simulink model "FMS1"  (R2018b)
settings: configuration reference "fms_config" (kept outside this file)
values from neighbouring files (symbols this model uses):
  FMS_EXPORT = Simulink.Parameter(FMS_EXPORT_VALUE)    [fms_model_init.m]
  FMS_PARAM = Simulink.Parameter(FMS_PARAM_VALUE)    [fms_model_init.m]
undefined symbols (not defined in the file or in its folder): actuator_cmd, ax_cmd, ay_cmd, az_cmd, cmd_mask, ControlMode, ctrl_mode, DiscIntNeverNeededParam, FMS_Cmd, FMS_CONST, home, mode, p_cmd, phi_cmd, PilotMode, psi_rate_cmd, q_cmd, r_cmd, reset, state, status, theta_cmd, throttle_cmd, timestamp, u_cmd, v_cmd, VehicleState, VehicleStatus, w_cmd, wp_consume, wp_current
libraries: simulink x119, FMT_Model_Lib x56, hdlsllib x13
(part 4 of 7)

== system FMS1/FMS Commander/Commander/Arm/Assist/Position/Position Command/Controller/Hold Control ==
  FMS_In : Inport
  Action Port : ActionPort  InitializeStates=reset  ActionType=case
  Bus Selector : BusSelector  OutputSignals=INS_Out.psi
  Bus_Selection : Subsystem
  Constant : Constant  Value=0  OutDataTypeStr=Inherit: Inherit via back propagation
  Delay : Delay  DelayLength=1  InitialConditionSource=Input port
      settings: InputPortMap=u0,p4
  Gain2 : Gain  Gain=FMS_PARAM.XY_P  OutDataTypeStr=single
  Multiply : Product  Multiplication=Matrix(*)
  Mux : Mux  Inputs=2
  Psi To DCM : FMT_Model_Lib/Transformation/Psi To DCM
      settings: SourceProductName=FMT Toolbox
  Selector : Selector  InputPortWidth=3  IndexOptions=Index vector (dialog)  Indices=[1 2]  OutputSizes=1
  Sum : Sum  Inputs=-+|
  uv_cmd_mPs : Outport
  wires:
  Bus Selector/1 -> Psi To DCM/1  "<psi>"
  Selector/1 -> Gain2/1
  Mux/1 -> Multiply/2
  Multiply/1 -> Selector/1
  Psi To DCM/1 -> Multiply/1  "M_CO"
  Constant/1 -> Mux/2
  FMS_In/1 -> Bus_Selection/1(FMS_In), Bus Selector/1
  Delay/1 -> Sum/2, Delay/1  "xy_cmd_R"
  Sum/1 -> Mux/1  "xy_err_R"
  Bus_Selection/1(xy_R_O_m) -> Delay/2, Sum/1  "xy_est_R"
  Gain2/1 -> uv_cmd_mPs/1

== system FMS1/FMS Commander/Commander/Arm/Assist/Position/Position Command/Controller/Move Control ==
  FMS_In : Inport
  Action Port : ActionPort  InitializeStates=reset  ActionType=case
  Bus Selector : BusSelector  OutputSignals=Pilot_Cmd.stick_pitch,Pilot_Cmd.stick_roll
  Compare To Constant : simulink/Logic and Bit Operations/Compare To Constant  relop=>  const=1  OutDataTypeStr=boolean
  DeadZone : Subsystem  mask{th=FMS_PARAM.PITCH_DZ}
      mask prompts: th "Threshold"
      mask Display: disp('Dead Zone')
  DeadZone1 : Subsystem  mask{th=FMS_PARAM.ROLL_DZ}
      mask prompts: th "Threshold"
      mask Display: disp('Dead Zone')
  Gain6 : Gain  Gain=FMS_PARAM.VEL_XY_LIM  OutDataTypeStr=single
  Mux1 : Mux  Inputs=2
  Switch : Switch  Criteria=u2 > Threshold
  TD : Subsystem
  Vector Modulus : FMT_Model_Lib/Math/Vector Modulus
      settings: SourceProductName=FMT Toolbox
  Vector Normalize : FMT_Model_Lib/Math/Vector Normalize
      settings: SourceProductName=FMT Toolbox
  uv_cmd_mPs : Outport
  wires:
  DeadZone1/1(y) -> Mux1/2
  Bus Selector/2 -> DeadZone1/1(u)  "<stick_roll>"
  TD/1(v1) -> uv_cmd_mPs/1
  FMS_In/1 -> Bus Selector/1
  Bus Selector/1 -> DeadZone/1(u)  "<stick_pitch>"
  DeadZone/1(y) -> Mux1/1
  Gain6/1 -> TD/1(v)
  Switch/1 -> Gain6/1
  Mux1/1 -> Switch/3, Vector Normalize/1, Vector Modulus/1
  Vector Modulus/1 -> Compare To Constant/1
  Compare To Constant/1 -> Switch/2
  Vector Normalize/1 -> Switch/1

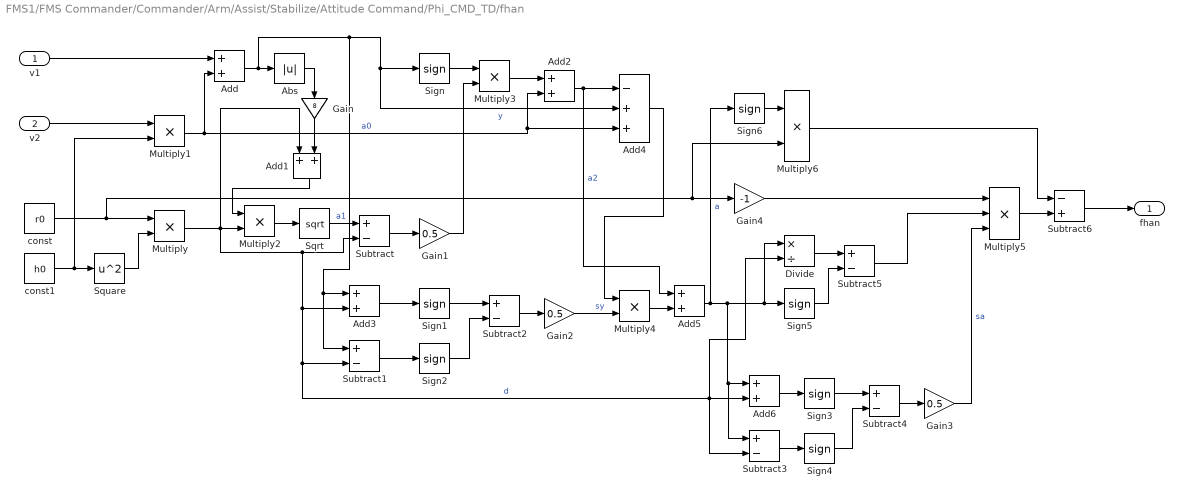
== system FMS1/FMS Commander/Commander/Arm/Assist/Stabilize/Attitude Command/Phi_CMD_TD/fhan  ==
  v1 : Inport
  v2 : Inport  Port=2
  Abs : Abs
  Add{,1..3,5..6} (6 alike) : Sum  OutDataTypeStr=Inherit: Same as first input
  Add4 : Sum  Inputs=-++
  Divide : Product  Inputs=*/
  Gain : Gain  Gain=8
  Gain1 : Gain  Gain=0.5  OutDataTypeStr=Inherit: Same as input
  Gain2 : Gain  Gain=0.5  OutDataTypeStr=Inherit: Same as input
  Gain3 : Gain  Gain=0.5  OutDataTypeStr=Inherit: Same as input
  Gain4 : Gain  Gain=-1  OutDataTypeStr=Inherit: Same as input
  Multiply{,1..3} (4 alike) : Product  OutDataTypeStr=Inherit: Same as first input
  Multiply4 : Product  OutDataTypeStr=single
  Multiply5 : Product  Inputs=3
  Multiply6 : Product  OutDataTypeStr=single
  Sign{,1..6} (7 alike) : Signum
  Sqrt : Sqrt  SaturateOnIntegerOverflow=on
  Square : Math  Operator=square  SaturateOnIntegerOverflow=on
  Subtract{,1..5} (6 alike) : Sum  Inputs=+-  OutDataTypeStr=Inherit: Same as first input
  Subtract6 : Sum  Inputs=-+  OutDataTypeStr=Inherit: Same as first input
  const : Constant  Value=r0  OutDataTypeStr=single
  const1 : Constant  Value=h0  OutDataTypeStr=single
  fhan : Outport
  wires:
  v1/1 -> Add/1
  Sign/1 -> Multiply3/1
  Gain2/1 -> Multiply4/2  "sy"
  v2/1 -> Multiply1/1
  Gain3/1 -> Multiply5/3  "sa"
  Subtract/1 -> Gain1/1
  Subtract6/1 -> fhan/1
  Sign2/1 -> Subtract2/2
  Sign4/1 -> Subtract4/2
  Abs/1 -> Gain/1
  Add4/1 -> Multiply4/1
  Sign5/1 -> Subtract5/2
  Sqrt/1 -> Subtract/1  "a1"
  Subtract3/1 -> Sign4/1
  Add1/1 -> Multiply2/1
  Subtract1/1 -> Sign2/1
  Divide/1 -> Subtract5/1
  Multiply3/1 -> Add2/1
  Gain/1 -> Add1/2
  const/1 -> Multiply6/2, Gain4/1, Multiply/1
  Add3/1 -> Sign1/1
  Subtract5/1 -> Multiply5/2
  Multiply4/1 -> Add5/2
  const1/1 -> Multiply1/2, Square/1
  Add5/1 -> Sign6/1, Sign5/1, Divide/1, Subtract3/1, Add6/1  "a"
  Multiply1/1 -> Add4/3, Add2/2, Add/2  "a0"
  Add/1 -> Subtract1/1, Add3/1, Add4/2, Sign/1, Abs/1  "y"
  Subtract2/1 -> Gain2/1
  Add2/1 -> Add4/1, Add5/1  "a2"
  Subtract4/1 -> Gain3/1
  Gain4/1 -> Multiply5/1
  Multiply5/1 -> Subtract6/2
  Sign6/1 -> Multiply6/1
  Sign3/1 -> Subtract4/1
  Add6/1 -> Sign3/1
  Multiply/1 -> Subtract/2, Divide/2, Subtract3/2, Add6/2, Subtract1/2, Add3/2, Add1/1, Multiply2/2  "d"
  Multiply6/1 -> Subtract6/1
  Gain1/1 -> Multiply3/2
  Square/1 -> Multiply/2
  Multiply2/1 -> Sqrt/1
  Sign1/1 -> Subtract2/1

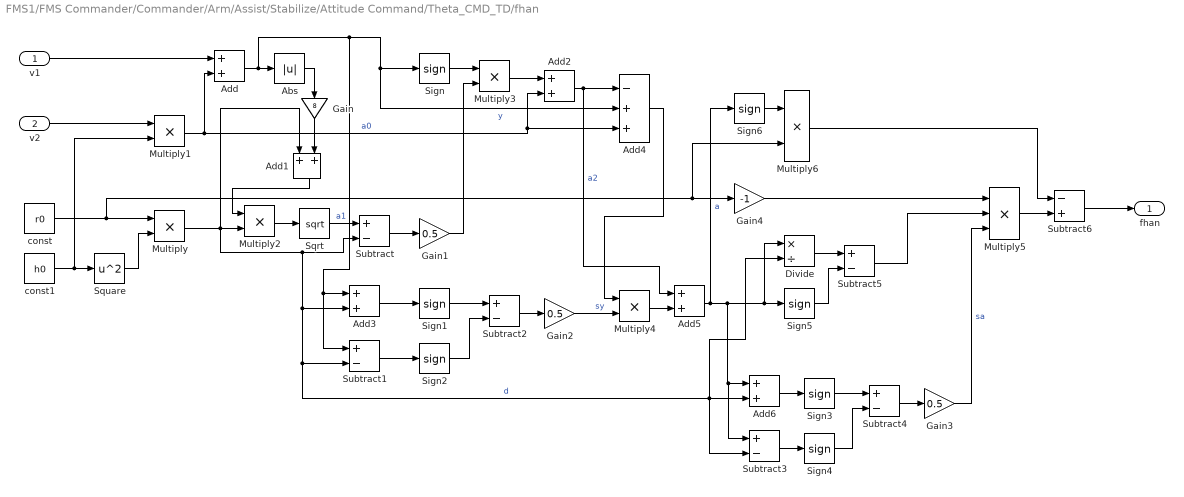
== system FMS1/FMS Commander/Commander/Arm/Assist/Stabilize/Attitude Command/Theta_CMD_TD/fhan  ==
  v1 : Inport
  v2 : Inport  Port=2
  Abs : Abs
  Add{,1..3,5..6} (6 alike) : Sum  OutDataTypeStr=Inherit: Same as first input
  Add4 : Sum  Inputs=-++
  Divide : Product  Inputs=*/
  Gain : Gain  Gain=8
  Gain1 : Gain  Gain=0.5  OutDataTypeStr=Inherit: Same as input
  Gain2 : Gain  Gain=0.5  OutDataTypeStr=Inherit: Same as input
  Gain3 : Gain  Gain=0.5  OutDataTypeStr=Inherit: Same as input
  Gain4 : Gain  Gain=-1  OutDataTypeStr=Inherit: Same as input
  Multiply{,1..3} (4 alike) : Product  OutDataTypeStr=Inherit: Same as first input
  Multiply4 : Product  OutDataTypeStr=single
  Multiply5 : Product  Inputs=3
  Multiply6 : Product  OutDataTypeStr=single
  Sign{,1..6} (7 alike) : Signum
  Sqrt : Sqrt  SaturateOnIntegerOverflow=on
  Square : Math  Operator=square  SaturateOnIntegerOverflow=on
  Subtract{,1..5} (6 alike) : Sum  Inputs=+-  OutDataTypeStr=Inherit: Same as first input
  Subtract6 : Sum  Inputs=-+  OutDataTypeStr=Inherit: Same as first input
  const : Constant  Value=r0  OutDataTypeStr=single
  const1 : Constant  Value=h0  OutDataTypeStr=single
  fhan : Outport
  wires:
  v1/1 -> Add/1
  Sign/1 -> Multiply3/1
  Gain2/1 -> Multiply4/2  "sy"
  v2/1 -> Multiply1/1
  Gain3/1 -> Multiply5/3  "sa"
  Subtract/1 -> Gain1/1
  Subtract6/1 -> fhan/1
  Sign2/1 -> Subtract2/2
  Sign4/1 -> Subtract4/2
  Abs/1 -> Gain/1
  Add4/1 -> Multiply4/1
  Sign5/1 -> Subtract5/2
  Sqrt/1 -> Subtract/1  "a1"
  Subtract3/1 -> Sign4/1
  Add1/1 -> Multiply2/1
  Subtract1/1 -> Sign2/1
  Divide/1 -> Subtract5/1
  Multiply3/1 -> Add2/1
  Gain/1 -> Add1/2
  const/1 -> Multiply6/2, Gain4/1, Multiply/1
  Add3/1 -> Sign1/1
  Subtract5/1 -> Multiply5/2
  Multiply4/1 -> Add5/2
  const1/1 -> Multiply1/2, Square/1
  Add5/1 -> Sign6/1, Sign5/1, Divide/1, Subtract3/1, Add6/1  "a"
  Multiply1/1 -> Add4/3, Add2/2, Add/2  "a0"
  Add/1 -> Subtract1/1, Add3/1, Add4/2, Sign/1, Abs/1  "y"
  Subtract2/1 -> Gain2/1
  Add2/1 -> Add4/1, Add5/1  "a2"
  Subtract4/1 -> Gain3/1
  Gain4/1 -> Multiply5/1
  Multiply5/1 -> Subtract6/2
  Sign6/1 -> Multiply6/1
  Sign3/1 -> Subtract4/1
  Add6/1 -> Sign3/1
  Multiply/1 -> Subtract/2, Divide/2, Subtract3/2, Add6/2, Subtract1/2, Add3/2, Add1/1, Multiply2/2  "d"
  Multiply6/1 -> Subtract6/1
  Gain1/1 -> Multiply3/2
  Square/1 -> Multiply/2
  Multiply2/1 -> Sqrt/1
  Sign1/1 -> Subtract2/1

== system FMS1/FMS Commander/Commander/Arm/Assist/Stabilize/Heading Command/Controller/Brake Control ==
  Action Port : ActionPort  InitializeStates=reset  ActionType=case
  Brake Speed : Constant  Value=0  VectorParams1D=off  OutDataTypeStr=single
  psi_rate_cmd_radPs : Outport
  wires:
  Brake Speed/1 -> psi_rate_cmd_radPs/1

== system FMS1/FMS Commander/Commander/Arm/Assist/Stabilize/Heading Command/Controller/Hold Control ==
  FMS_In : Inport
  Action Port : ActionPort  InitializeStates=reset  ActionType=case
  Bus_Selection : Subsystem
  Delay : Delay  DelayLength=1  InitialConditionSource=Input port
      settings: InputPortMap=u0,p4
  Gain2 : Gain  Gain=FMS_PARAM.YAW_P  OutDataTypeStr=single
  Sum : Sum  Inputs=-+|
  psi_err_saturation : Subsystem
  psi_rate_cmd_radPs : Outport
  wires:
  Gain2/1 -> psi_rate_cmd_radPs/1
  FMS_In/1 -> Bus_Selection/1(FMS_In)
  Delay/1 -> Sum/2, Delay/1  "psi_cmd_rad"
  Sum/1 -> psi_err_saturation/1(psi_err_in)  "psi_error_rad"
  psi_err_saturation/1(psi_err_rad) -> Gain2/1
  Bus_Selection/1(psi_rad) -> Delay/2, Sum/1  "psi_est_rad"

== system FMS1/FMS Commander/Commander/Arm/Assist/Stabilize/Heading Command/Controller/Move Control ==
  FMS_In : Inport
  Action Port : ActionPort  InitializeStates=reset  ActionType=case
  Bus Selector : BusSelector  OutputSignals=Pilot_Cmd.stick_yaw
  DeadZone : Subsystem  mask{th=FMS_PARAM.YAW_DZ}
      mask prompts: th "Threshold"
      mask Display: disp('Dead Zone')
  Gain1 : Gain  Gain=FMS_PARAM.YAW_RATE_LIM  OutDataTypeStr=single
  TD : Subsystem
  psi_rate_cmd_radPs : Outport
  wires:
  TD/1(v1) -> psi_rate_cmd_radPs/1
  FMS_In/1 -> Bus Selector/1
  Bus Selector/1 -> DeadZone/1(u)  "<stick_yaw>"
  DeadZone/1(y) -> Gain1/1
  Gain1/1 -> TD/1(v)

== system FMS1/FMS Commander/Commander/Arm/Auto/Mission/Mission_SubSystem/Heading Commander/Heading Control ==
  FMS_In : Inport
  psi_cmd_rad : Inport  Port=2
  Bus Selector : BusSelector  OutputSignals=INS_Out.psi
  Delay : Delay  DelayLength=1  InitialConditionSource=Input port
      settings: InputPortMap=u0,p4
  Heading Control : Subsystem
  Sum : Sum  Inputs=|++
  Sum1 : Sum  Inputs=+-|
  Sum2 : Sum  Inputs=|+-
  TD : Subsystem
  psi_saturation : Subsystem
  psi_saturation1 : Subsystem
  psi_rate_cmd_radPs : Outport
  psi_err_rad : Outport  Port=2
  wires:
  psi_cmd_rad/1 -> Sum2/1, Sum1/1
  Heading Control/1(psi_rate_cmd_radPs) -> psi_rate_cmd_radPs/1
  FMS_In/1 -> Heading Control/1(FMS_In), Bus Selector/1
  TD/1(v1) -> Heading Control/2(psi_cmd_rad)
  Sum1/1 -> psi_saturation1/1(psi_in)
  Bus Selector/1 -> Sum1/2, Delay/2  "<psi>"
  psi_saturation1/1(psi_rad) -> psi_err_rad/1
  Delay/1 -> Delay/1, TD/2(v0), Sum/2, Sum2/2
  Sum2/1 -> psi_saturation/1(psi_in)
  psi_saturation/1(psi_rad) -> Sum/1
  Sum/1 -> TD/1(v)

== system FMS1/FMS Commander/Commander/Arm/Auto/Mission/Mission_SubSystem/Heading Commander/Included Angle ==
  vec1 : Inport
  vec2 : Inport  Port=2
  2D Cross Product : FMT_Model_Lib/Math/2D Cross Product
      settings: SourceProductName=FMT Toolbox
  Acos : Trigonometry  Operator=acos
  Constant4 : Constant  OutDataTypeStr=single
  Demux : Demux  Outputs=2
  Demux1 : Demux  Outputs=2
  Dot Product : DotProduct  InputSameDT=on  OutDataTypeStr=Inherit: Inherit via internal rule
  Multiply : Product
  Mux : Mux  Inputs=2
  Mux1 : Mux  Inputs=2
  Sign1 : Signum
  Switch2 : Switch  Criteria=u2 ~= 0
  Vector Normalize : FMT_Model_Lib/Math/Vector Normalize
      settings: SourceProductName=FMT Toolbox
  Vector Normalize1 : FMT_Model_Lib/Math/Vector Normalize
      settings: SourceProductName=FMT Toolbox
  angle_rad : Outport
  wires:
  Switch2/1 -> Multiply/2
  Acos/1 -> Multiply/1
  Mux/1 -> Vector Normalize1/1
  vec2/1 -> Demux/1
  Constant4/1 -> Switch2/3
  Demux/1 -> Mux/2
  vec1/1 -> Demux1/1
  Multiply/1 -> angle_rad/1
  2D Cross Product/1 -> Sign1/1
  Vector Normalize/1 -> 2D Cross Product/2, Dot Product/1
  Demux/2 -> Mux/1
  Vector Normalize1/1 -> 2D Cross Product/1, Dot Product/2
  Sign1/1 -> Switch2/2, Switch2/1
  Demux1/2 -> Mux1/1
  Mux1/1 -> Vector Normalize/1
  Demux1/1 -> Mux1/2
  Dot Product/1 -> Acos/1

== system FMS1/FMS Commander/Commander/Arm/Auto/Mission/Mission_SubSystem/Velocity Commander/Altitude Control ==
  FMS_In : Inport
  Vg_C_cmd : Inport  Port=2
  Bus Selector3 : BusSelector  OutputSignals=INS_Out.h_R
  Gain : Gain  Gain=FMS_PARAM.Z_P
  Mux : Mux  Inputs=2
  Saturation1 : Saturate  UpperLimit=FMS_PARAM.VEL_Z_LIM  LowerLimit=-FMS_PARAM.VEL_Z_LIM
  Selector : Selector  InputPortWidth=3  IndexOptions=Index vector (dialog)  Indices=[1 2]  OutputSizes=1
  Sum2 : Sum  Inputs=|+-
  Target Height : Subsystem
  vel_C_cmd : Outport
  wires:
  FMS_In/1 -> Bus Selector3/1, Target Height/1(FMS_In)
  Bus Selector3/1 -> Sum2/1  "<h_R>"
  Sum2/1 -> Gain/1
  Gain/1 -> Saturation1/1
  Target Height/1(h_R_sp) -> Sum2/2  "h_R_sp"
  Vg_C_cmd/1 -> Selector/1
  Selector/1 -> Mux/1
  Saturation1/1 -> Mux/2
  Mux/1 -> vel_C_cmd/1

== system FMS1/FMS Commander/Commander/Arm/Auto/Mission/Mission_SubSystem/Velocity Commander/Cruise Speed  ==
  P3 : Inport
  P2 : Inport  Port=2
  set_speed : Inport  Port=3
  rotating : Inport  Port=4
  Acceleration_Speed : DiscreteIntegrator  ExternalReset=level  SampleTime=-1  UpperSaturationLimit=FMS_PARAM.CRUISE_SPEED  LowerSaturationLimit=0  ICPrevOutput=DiscIntNeverNeededParam  ICPrevScaledInput=DiscIntNeverNeededParam
  Compare To Zero : simulink/Logic and Bit Operations/Compare To Zero  relop=>  OutDataTypeStr=boolean
  Constant : Constant  Value=FMS_PARAM.CRUISE_ACC  OutDataTypeStr=single
  Constant1 : Constant  Value=0.5  OutDataTypeStr=single
  Constant2 : Constant  Value=0  OutDataTypeStr=single
  Gain : Gain  Gain=0.5  OutDataTypeStr=Inherit: Same as input
  Saturation Dynamic : simulink/Discontinuities/Saturation Dynamic  OutMin=[]  OutMax=[]  OutDataTypeStr=Inherit: Same as second input  OutDataType=fixdt(1, 16)  OutScaling=2^-10  DoSatur=off
  Saturation Dynamic1 : simulink/Discontinuities/Saturation Dynamic  OutMin=[]  OutMax=[]  OutDataTypeStr=Inherit: Same as second input  OutDataType=fixdt(1, 16)  OutScaling=2^-10  DoSatur=off
  Sum : Sum  Inputs=|+-
  Sum1 : Sum  Inputs=-+|
  Switch : Switch  Criteria=u2 > Threshold  Threshold=FMS_PARAM.L1
  Switch1 : Switch
  Switch2 : Switch  Criteria=u2 > Threshold
  Vector Modulus : FMT_Model_Lib/Math/Vector Modulus
      settings: SourceProductName=FMT Toolbox
  vel : Constant  Value=FMS_PARAM.CRUISE_SPEED  OutDataTypeStr=single
  |Vg| : Outport
  cruise_speed : Outport  Port=2
  wires:
  Gain/1 -> Saturation Dynamic/2
  Switch/1 -> Sum1/1, Switch1/1
  vel/1 -> Switch2/3  "|Vg|"
  Vector Modulus/1 -> Switch/2, Gain/1
  Sum/1 -> Vector Modulus/1
  P2/1 -> Sum/2
  P3/1 -> Sum/1
  Saturation Dynamic/1 -> Switch/3
  Constant/1 -> Acceleration_Speed/1
  Saturation Dynamic1/1 -> Switch1/3, Sum1/2
  Sum1/1 -> Switch1/2
  Switch1/1 -> |Vg|/1
  rotating/1 -> Acceleration_Speed/2
  Switch2/1 -> cruise_speed/1, Saturation Dynamic1/1, Saturation Dynamic/1, Switch/1
  set_speed/1 -> Compare To Zero/1, Switch2/1
  Compare To Zero/1 -> Switch2/2
  Constant1/1 -> Saturation Dynamic/3
  Acceleration_Speed/1 -> Saturation Dynamic1/2
  Constant2/1 -> Saturation Dynamic1/3

== system FMS1/FMS Commander/Commander/Arm/Auto/Mission/Mission_SubSystem/Velocity Commander/Hold Position ==
  FMS_In : Inport
  Altitude Hold : Subsystem
  Mux : Mux  Inputs=3
  Position Hold : Subsystem
  vel_cmd : Outport
  wires:
  FMS_In/1 -> Altitude Hold/1(FMS_In), Position Hold/1(FMS_In)
  Position Hold/2(v_cmd_mPs) -> Mux/2
  Altitude Hold/1(w_cmd_mPs) -> Mux/3
  Position Hold/1(u_cmd_mPs) -> Mux/1
  Mux/1 -> vel_cmd/1

== system FMS1/FMS Commander/Commander/Arm/Auto/Mission/Mission_SubSystem/Velocity Commander/L1 Reference WP ==
  P1 : Inport
  P2 : Inport  Port=2
  P3 : Inport  Port=3
  L1 : Inport  Port=4
  Compare To Constant : simulink/Logic and Bit Operations/Compare To Constant  relop=>=  const=0  OutDataTypeStr=boolean
  Compare To Constant1 : simulink/Logic and Bit Operations/Compare To Constant  relop=>  const=0  OutDataTypeStr=boolean
  NearbyRefWP : MATLAB Function  TreatAsAtomicUnit=on
  OutRegionRegWP : MATLAB Function  TreatAsAtomicUnit=on
  Reshape : Reshape  OutputDimensionality=Customize  OutputDimensions=[2,1]
  SearchL1RefWP : MATLAB Function  TreatAsAtomicUnit=on
  Switch : Switch  Criteria=u2 > Threshold
  Switch1 : Switch  Criteria=u2 > Threshold
  L1_WP : Outport
  wires:
  Reshape/1 -> L1_WP/1
  Compare To Constant/1 -> Switch/2
  NearbyRefWP/2(d) -> Compare To Constant1/1  "distance"
  SearchL1RefWP/2(u) -> Compare To Constant/1  "l1_u"
  Compare To Constant1/1 -> Switch1/2
  P1/1 -> SearchL1RefWP/1(P1), OutRegionRegWP/1(P1)
  P2/1 -> SearchL1RefWP/2(P2), NearbyRefWP/1(P2), OutRegionRegWP/2(P2)
  P3/1 -> NearbyRefWP/2(P3), SearchL1RefWP/3(P3), OutRegionRegWP/3(P3)
  Switch/1 -> Switch1/3
  L1/1 -> SearchL1RefWP/4(L1), NearbyRefWP/3(L1)
  OutRegionRegWP/1(P) -> Switch/3  "out_WP"
  Switch1/1 -> Reshape/1
  SearchL1RefWP/1(P) -> Switch/1  "L1_Ref_P"
  NearbyRefWP/1(P) -> Switch1/1  "NearbyWP"

== system FMS1/FMS Commander/Commander/Arm/Auto/Mission/Mission_SubSystem/Velocity Commander/Lateral Acceleration ==
  Vg : Inport
  L1_WP : Inport  Port=2
  p3 : Inport  Port=3
  L1 : Inport  Port=4
  Constant : Constant  Value=0.5  OutDataTypeStr=Inherit: Inherit via back propagation
  Divide : Product  Inputs=*/
  Gain : Gain  Gain=2
  Included Angle : Subsystem
  Max : MinMax  Function=max  Inputs=2
  Min : MinMax  Inputs=2
  Multiply1 : Product
  Saturation : Saturate  UpperLimit=pi/2  LowerLimit=-pi/2
  Sin : Trigonometry
  Square : Math  Operator=square  SaturateOnIntegerOverflow=on
  Subtract : Sum  Inputs=+-
  Vector Modulus : FMT_Model_Lib/Math/Vector Modulus
      settings: SourceProductName=FMT Toolbox
  Vector Modulus1 : FMT_Model_Lib/Math/Vector Modulus
      settings: SourceProductName=FMT Toolbox
  Vector Normalize : FMT_Model_Lib/Math/Vector Normalize
      settings: SourceProductName=FMT Toolbox
  Vector Normalize1 : FMT_Model_Lib/Math/Vector Normalize
      settings: SourceProductName=FMT Toolbox
  l1_a_cmd : Outport
  wires:
  Saturation/1 -> Sin/1
  Included Angle/1(angle_rad) -> Saturation/1  "L1_alpha"
  Vector Modulus/1 -> Square/1
  Subtract/1 -> Vector Modulus1/1, Vector Normalize1/1
  Gain/1 -> Multiply1/2
  L1_WP/1 -> Subtract/1
  Vector Normalize/1 -> Included Angle/1(vec1)
  Multiply1/1 -> Divide/1
  Divide/1 -> l1_a_cmd/1  "l1_a_cmd"
  Vector Normalize1/1 -> Included Angle/2(vec2)
  Square/1 -> Gain/1
  L1/1 -> Min/1
  Vg/1 -> Vector Normalize/1, Vector Modulus/1
  Sin/1 -> Multiply1/1  "sin_alpha"
  p3/1 -> Subtract/2
  Vector Modulus1/1 -> Max/1
  Constant/1 -> Max/2
  Max/1 -> Min/2
  Min/1 -> Divide/2

== system FMS1/FMS Commander/Commander/Arm/Auto/Mission/Mission_SubSystem/Velocity Commander/Lateral Acceleration To Speed ==
  l1_a : Inport
  p3 : Inport  Port=2
  p2 : Inport  Port=3
  |Vg| : Inport  Port=4
  cruise_speed : Inport  Port=5
  psi : Inport  Port=6
  Delay : Delay  DelayLength=1  InitialConditionSource=Input port
      settings: InputPortMap=u0,p4
  Divide1 : Product  Inputs=*/
  Ground Speed : Subsystem
  Multiply : Product  Multiplication=Matrix(*)
  Rotation Matrix : Subsystem
  Saturation : Saturate  UpperLimit=pi/10  LowerLimit=-pi/10
  Sum : Sum  Inputs=|+-
  Vg_C_cmd : Outport
  wires:
  psi/1 -> Rotation Matrix/2(psi)
  Sum/1 -> Ground Speed/2(p3p2)
  p2/1 -> Sum/1
  l1_a/1 -> Divide1/1
  |Vg|/1 -> Ground Speed/1(|Vg|)
  p3/1 -> Delay/2
  Multiply/1 -> Vg_C_cmd/1
  Rotation Matrix/1(M_CO) -> Multiply/1
  Divide1/1 -> Saturation/1
  Ground Speed/1(Vg_O_cmd) -> Multiply/2
  Delay/1 -> Delay/1, Sum/2
  Saturation/1 -> Rotation Matrix/1(l1_omega)
  cruise_speed/1 -> Divide1/2

== system FMS1/FMS Commander/Commander/Arm/Auto/Mission/Mission_SubSystem/Velocity Commander/ValidCounter ==
  in : Inport
  Compare To Constant : simulink/Logic and Bit Operations/Compare To Constant  relop=>  const=3.0  OutDataTypeStr=boolean
  Discrete-Time Integrator : DiscreteIntegrator  IntegratorMethod=Accumulation: Forward Euler  SampleTime=-1  LimitOutput=on  UpperSaturationLimit=100  LowerSaturationLimit=0  ICPrevOutput=DiscIntNeverNeededParam  ICPrevScaledInput=DiscIntNeverNeededParam
  out : Outport
  wires:
  in/1 -> Discrete-Time Integrator/1
  Discrete-Time Integrator/1 -> Compare To Constant/1
  Compare To Constant/1 -> out/1

== system FMS1/FMS Commander/Commander/Arm/Auto/Offboard/Heading_Command/Heading_Control/Error ==
  FMS_In : Inport
  Bus Selector3 : BusSelector  OutputSignals=INS_Out.psi
  Bus Selector4 : BusSelector  OutputSignals=Auto_Cmd.psi_cmd
  Constant : Constant  Value=2*pi  OutDataTypeStr=single
  Math Function : Math  Operator=rem  SaturateOnIntegerOverflow=on
  Saturation : Saturate  UpperLimit=pi/10  LowerLimit=-pi/10
  Sum1 : Sum  Inputs=-+|
  psi_err_saturation : Subsystem
  psi_error : Outport
  wires:
  psi_err_saturation/1(psi_err_rad) -> Saturation/1
  Sum1/1 -> psi_err_saturation/1(psi_err_in)
  FMS_In/1 -> Bus Selector3/1, Bus Selector4/1
  Bus Selector3/1 -> Sum1/1  "<psi>"
  Bus Selector4/1 -> Math Function/1  "<psi_cmd>"
  Math Function/1 -> Sum1/2
  Constant/1 -> Math Function/2
  Saturation/1 -> psi_error/1

== system FMS1/FMS Commander/Commander/Arm/Auto/Offboard/Velocity_Command/Position_Control/Body_Error ==
  psi : Inport
  pos_est_O : Inport  Port=2
  pos_C_cmd : Inport  Port=3
  pos_mask : Inport  Port=4
  Multiply : Product
  Multiply2 : Product  Multiplication=Matrix(*)
  Psi To DCM1 : FMT_Model_Lib/Transformation/Psi To DCM
      settings: SourceProductName=FMT Toolbox
  Saturation1 : Saturate  UpperLimit=[4,4,2]  LowerLimit=[-4,-4,-2]
  Sum2 : Sum  Inputs=+-|
  pos_error_C : Outport
  wires:
  Multiply2/1 -> Sum2/2
  pos_C_cmd/1 -> Sum2/1
  Sum2/1 -> Multiply/1
  pos_est_O/1 -> Multiply2/2
  Saturation1/1 -> pos_error_C/1
  Psi To DCM1/1 -> Multiply2/1  "M_CO"
  psi/1 -> Psi To DCM1/1
  pos_mask/1 -> Multiply/2
  Multiply/1 -> Saturation1/1

== system FMS1/FMS Commander/Commander/Arm/Auto/Offboard/Velocity_Command/Position_Control/Command_Mask ==
  FMS_In : Inport
  Bus Selector3 : BusSelector  OutputSignals=Auto_Cmd.cmd_mask
  Compare To Zero : simulink/Logic and Bit Operations/Compare To Zero  relop=>  OutDataTypeStr=boolean
  Compare To Zero1 : simulink/Logic and Bit Operations/Compare To Zero  relop=>  OutDataTypeStr=boolean
  Logical Operator : Logic  Operator=OR  AllPortsSameDT=off  OutDataTypeStr=boolean
  Mux : Mux  Inputs=3
  Mux3 : Mux  Inputs=3
  alt_cmd valid : simulink/Logic and Bit Operations/Bitwise Operator  logicop=AND  UseBitMask=on  BitMask=bin2dec('1000000000000')  BitMaskRealWorld=Stored Integer
  lat_cmd valid : simulink/Logic and Bit Operations/Bitwise Operator  logicop=AND  UseBitMask=on  BitMask=bin2dec('10000000000')  BitMaskRealWorld=Stored Integer
  lon_cmd valid : simulink/Logic and Bit Operations/Bitwise Operator  logicop=AND  UseBitMask=on  BitMask=bin2dec('100000000000')  BitMaskRealWorld=Stored Integer
  x_cmd valid : simulink/Logic and Bit Operations/Bitwise Operator  logicop=AND  UseBitMask=on  BitMask=bin2dec('10000000')  BitMaskRealWorld=Stored Integer
  y_cmd valid : simulink/Logic and Bit Operations/Bitwise Operator  logicop=AND  UseBitMask=on  BitMask=bin2dec('100000000')  BitMaskRealWorld=Stored Integer
  z_cmd valid : simulink/Logic and Bit Operations/Bitwise Operator  logicop=AND  UseBitMask=on  BitMask=bin2dec('1000000000')  BitMaskRealWorld=Stored Integer
  pos_mask : Outport
  wires:
  FMS_In/1 -> Bus Selector3/1
  x_cmd valid/1 -> Mux/1
  z_cmd valid/1 -> Mux/3
  y_cmd valid/1 -> Mux/2
  Mux/1 -> Compare To Zero/1
  lon_cmd valid/1 -> Mux3/2
  alt_cmd valid/1 -> Mux3/3
  Mux3/1 -> Compare To Zero1/1
  lat_cmd valid/1 -> Mux3/1
  Bus Selector3/1 -> y_cmd valid/1, x_cmd valid/1, z_cmd valid/1, lat_cmd valid/1, lon_cmd valid/1, alt_cmd valid/1  "<cmd_mask>"
  Compare To Zero1/1 -> Logical Operator/2
  Compare To Zero/1 -> Logical Operator/1
  Logical Operator/1 -> pos_mask/1

== system FMS1/FMS Commander/Commander/Arm/Auto/Offboard/Velocity_Command/Position_Control/Global_Error ==
  psi : Inport
  pos_est_O : Inport  Port=2
  pos_O_cmd : Inport  Port=3
  pos_mask : Inport  Port=4
  Multiply : Product
  Multiply1 : Product  Multiplication=Matrix(*)
  Psi To DCM : FMT_Model_Lib/Transformation/Psi To DCM
      settings: SourceProductName=FMT Toolbox
  Saturation : Saturate  UpperLimit=[4,4,2]  LowerLimit=[-4,-4,-2]
  Sum1 : Sum  Inputs=-+|
  pos_error_C : Outport
  wires:
  pos_est_O/1 -> Sum1/1
  Psi To DCM/1 -> Multiply1/1  "M_CO"
  Multiply1/1 -> pos_error_C/1
  psi/1 -> Psi To DCM/1
  pos_O_cmd/1 -> Sum1/2
  Saturation/1 -> Multiply1/2
  Sum1/1 -> Multiply/1
  pos_mask/1 -> Multiply/2
  Multiply/1 -> Saturation/1

== system FMS1/FMS Commander/Commander/Arm/Auto/Offboard/Velocity_Command/Position_Control/Local_Error ==
  psi : Inport
  psi_0 : Inport  Port=2
  pos_est_O : Inport  Port=3
  pos_R_cmd : Inport  Port=4
  pos_mask : Inport  Port=5
  Multiply : Product
  Multiply2 : Product  Multiplication=Matrix(*)
  Multiply3 : Product  Multiplication=Matrix(*)
  Psi To DCM1 : FMT_Model_Lib/Transformation/Psi To DCM
      settings: SourceProductName=FMT Toolbox
  Psi To DCM2 : FMT_Model_Lib/Transformation/Psi To DCM
      settings: SourceProductName=FMT Toolbox
  Saturation1 : Saturate  UpperLimit=[4,4,2]  LowerLimit=[-4,-4,-2]
  Subtract : Sum  Inputs=+-
  Sum2 : Sum  Inputs=+-|
  pos_error_C : Outport
  wires:
  Psi To DCM1/1 -> Multiply2/1  "M_RO"
  Multiply3/1 -> pos_error_C/1
  pos_est_O/1 -> Multiply2/2
  psi/1 -> Subtract/1
  pos_R_cmd/1 -> Sum2/1
  Saturation1/1 -> Multiply3/2
  Multiply2/1 -> Sum2/2
  Subtract/1 -> Psi To DCM2/1
  psi_0/1 -> Subtract/2, Psi To DCM1/1  "psi_0"
  Psi To DCM2/1 -> Multiply3/1  "M_CR"
  Sum2/1 -> Multiply/1
  pos_mask/1 -> Multiply/2
  Multiply/1 -> Saturation1/1

== system FMS1/FMS Commander/Commander/Arm/Auto/Offboard/Velocity_Command/Position_Control/Position_Command ==
  FMS_In : Inport
  Command_Mask : Subsystem
  Global_Position_Command : Subsystem
  Local_Position_Command : Subsystem
  Switch : Switch  Criteria=u2 > Threshold
  pos_cmd_O : Outport
  wires:
  FMS_In/1 -> Local_Position_Command/1(FMS_In), Command_Mask/1(FMS_In), Global_Position_Command/1(FMS_In)
  Switch/1 -> pos_cmd_O/1
  Local_Position_Command/1(pos_cmd_O) -> Switch/3
  Global_Position_Command/1(pos_cmd_O) -> Switch/1
  Command_Mask/1(global_cmd_valid) -> Switch/2

== system FMS1/FMS Commander/Commander/Arm/Auto/Offboard/Velocity_Command/Position_Control/Position_State ==
  FMS_In : Inport
  Bus Selector3 : BusSelector  OutputSignals=INS_Out.x_R,INS_Out.y_R,INS_Out.h_R
  Gain : Gain  Gain=-1
  Mux1 : Mux  Inputs=3
  pos_est_O : Outport
  wires:
  Bus Selector3/2 -> Mux1/2  "<y_R>"
  FMS_In/1 -> Bus Selector3/1
  Bus Selector3/3 -> Gain/1  "<h_R>"
  Mux1/1 -> pos_est_O/1  "pos_est"
  Gain/1 -> Mux1/3
  Bus Selector3/1 -> Mux1/1  "<x_R>"

== system FMS1/FMS Commander/Commander/Arm/Auto/Offboard/Velocity_Command/Velocity_Command/Body_Frame ==
  vel_cmd_B : Inport
  vel_cmd_C : Outport
  wires:
  vel_cmd_B/1 -> vel_cmd_C/1

== system FMS1/FMS Commander/Commander/Arm/Auto/Offboard/Velocity_Command/Velocity_Command/Command_Mask ==
  FMS_In : Inport
  Bus Selector1 : BusSelector  OutputSignals=Auto_Cmd.cmd_mask
  Compare To Zero2 : simulink/Logic and Bit Operations/Compare To Zero  relop=>  OutDataTypeStr=boolean
  Mux : Mux  Inputs=3
  u_cmd valid : simulink/Logic and Bit Operations/Bitwise Operator  logicop=AND  UseBitMask=on  BitMask=bin2dec('10000000000000')  BitMaskRealWorld=Stored Integer
  v_cmd valid : simulink/Logic and Bit Operations/Bitwise Operator  logicop=AND  UseBitMask=on  BitMask=bin2dec('100000000000000')  BitMaskRealWorld=Stored Integer
  w_cmd valid : simulink/Logic and Bit Operations/Bitwise Operator  logicop=AND  UseBitMask=on  BitMask=bin2dec('1000000000000000')  BitMaskRealWorld=Stored Integer
  vel_mask : Outport
  wires:
  w_cmd valid/1 -> Mux/3
  Compare To Zero2/1 -> vel_mask/1
  u_cmd valid/1 -> Mux/1
  v_cmd valid/1 -> Mux/2
  FMS_In/1 -> Bus Selector1/1
  Mux/1 -> Compare To Zero2/1
  Bus Selector1/1 -> w_cmd valid/1, v_cmd valid/1, u_cmd valid/1  "<cmd_mask>"

== system FMS1/FMS Commander/Commander/Arm/Auto/Offboard/Velocity_Command/Velocity_Command/Global_Frame ==
  psi : Inport
  vel_cmd_O : Inport  Port=2
  Multiply : Product  Multiplication=Matrix(*)
  Psi To DCM : FMT_Model_Lib/Transformation/Psi To DCM
      settings: SourceProductName=FMT Toolbox
  vel_cmd_C : Outport
  wires:
  psi/1 -> Psi To DCM/1
  Psi To DCM/1 -> Multiply/1  "M_CO"
  vel_cmd_O/1 -> Multiply/2
  Multiply/1 -> vel_cmd_C/1

== system FMS1/FMS Commander/Commander/Arm/Auto/Offboard/Velocity_Command/Velocity_Command/Local_Frame ==
  psi : Inport
  psi_0 : Inport  Port=2
  vel_cmd_R : Inport  Port=3
  Multiply3 : Product  Multiplication=Matrix(*)
  Psi To DCM2 : FMT_Model_Lib/Transformation/Psi To DCM
      settings: SourceProductName=FMT Toolbox
  Subtract : Sum  Inputs=+-
  vel_cmd_C : Outport
  wires:
  Psi To DCM2/1 -> Multiply3/1  "M_CR"
  Subtract/1 -> Psi To DCM2/1
  psi/1 -> Subtract/1
  vel_cmd_R/1 -> Multiply3/2
  Multiply3/1 -> vel_cmd_C/1
  psi_0/1 -> Subtract/2

== system FMS1/FMS Commander/Commander/Arm/SubMode/Hold/Altitude Hold/Controller/Brake Control ==
  Action Port : ActionPort  InitializeStates=reset  ActionType=case
  Brake Speed : Constant  Value=0  VectorParams1D=off  OutDataTypeStr=single
  psi_rate_cmd_radPs : Outport
  wires:
  Brake Speed/1 -> psi_rate_cmd_radPs/1

== system FMS1/FMS Commander/Commander/Arm/SubMode/Hold/Altitude Hold/Controller/Hold Control ==
  FMS_In : Inport
  Action Port : ActionPort  InitializeStates=reset  ActionType=case
  Bus_Selection : Subsystem
  Delay : Delay  DelayLength=1  InitialConditionSource=Input port
      settings: InputPortMap=u0,p4
  Gain2 : Gain  Gain=FMS_PARAM.Z_P  OutDataTypeStr=single
  Sum : Sum  Inputs=-+|
  w_cmd_mPs : Outport
  wires:
  FMS_In/1 -> Bus_Selection/1(FMS_In)
  Delay/1 -> Sum/2, Delay/1  "z_cmd_R"
  Sum/1 -> Gain2/1  "z_err_R"
  Bus_Selection/1(z_R_m) -> Delay/2, Sum/1  "z_est_R"
  Gain2/1 -> w_cmd_mPs/1

== system FMS1/FMS Commander/Commander/Arm/SubMode/Hold/Altitude Hold/Controller/Move Control ==
  FMS_In : Inport
  Action Port : ActionPort  InitializeStates=reset  ActionType=case
  Bus Selector : BusSelector  OutputSignals=Pilot_Cmd.stick_throttle
  DeadZone : Subsystem  mask{th=FMS_PARAM.THROTTLE_DZ}
      mask prompts: th "Threshold"
      mask Display: disp('Dead Zone')
  Gain1 : Gain  Gain=-FMS_PARAM.VEL_Z_LIM  OutDataTypeStr=single
  TD1 : Subsystem
  w_cmd_mPs : Outport
  wires:
  TD1/1(v1) -> w_cmd_mPs/1
  FMS_In/1 -> Bus Selector/1
  Bus Selector/1 -> DeadZone/1(u)  "<stick_throttle>"
  DeadZone/1(y) -> Gain1/1
  Gain1/1 -> TD1/1(v)

== system FMS1/FMS Commander/Commander/Arm/SubMode/Hold/Heading Hold/Controller/Brake Control ==
  Action Port : ActionPort  InitializeStates=reset  ActionType=case
  Brake Speed : Constant  Value=0  VectorParams1D=off  OutDataTypeStr=single
  psi_rate_cmd_radPs : Outport
  wires:
  Brake Speed/1 -> psi_rate_cmd_radPs/1

== system FMS1/FMS Commander/Commander/Arm/SubMode/Hold/Heading Hold/Controller/Hold Control ==
  FMS_In : Inport
  Action Port : ActionPort  InitializeStates=reset  ActionType=case
  Bus_Selection : Subsystem
  Delay : Delay  DelayLength=1  InitialConditionSource=Input port
      settings: InputPortMap=u0,p4
  Gain2 : Gain  Gain=FMS_PARAM.YAW_P  OutDataTypeStr=single
  Sum : Sum  Inputs=-+|
  psi_err_saturation : Subsystem
  psi_rate_cmd_radPs : Outport
  wires:
  Gain2/1 -> psi_rate_cmd_radPs/1
  FMS_In/1 -> Bus_Selection/1(FMS_In)
  Delay/1 -> Sum/2, Delay/1  "psi_cmd_rad"
  Sum/1 -> psi_err_saturation/1(psi_err_in)  "psi_error_rad"
  psi_err_saturation/1(psi_err_rad) -> Gain2/1
  Bus_Selection/1(psi_rad) -> Delay/2, Sum/1  "psi_est_rad"

== system FMS1/FMS Commander/Commander/Arm/SubMode/Hold/Heading Hold/Controller/Move Control ==
  FMS_In : Inport
  Action Port : ActionPort  InitializeStates=reset  ActionType=case
  Bus Selector : BusSelector  OutputSignals=Pilot_Cmd.stick_yaw
  DeadZone : Subsystem  mask{th=FMS_PARAM.YAW_DZ}
      mask prompts: th "Threshold"
      mask Display: disp('Dead Zone')
  Gain1 : Gain  Gain=FMS_PARAM.YAW_RATE_LIM  OutDataTypeStr=single
  TD : Subsystem
  psi_rate_cmd_radPs : Outport
  wires:
  TD/1(v1) -> psi_rate_cmd_radPs/1
  FMS_In/1 -> Bus Selector/1
  Bus Selector/1 -> DeadZone/1(u)  "<stick_yaw>"
  DeadZone/1(y) -> Gain1/1
  Gain1/1 -> TD/1(v)

== system FMS1/FMS Commander/Commander/Arm/SubMode/Hold/Position Hold/Controller/Brake Control ==
  Action Port : ActionPort  InitializeStates=reset  ActionType=case
  Brake Speed : Constant  Value=[0;0]  VectorParams1D=off  OutDataTypeStr=single
  uv_cmd_mPs : Outport
  wires:
  Brake Speed/1 -> uv_cmd_mPs/1

== system FMS1/FMS Commander/Commander/Arm/SubMode/Hold/Position Hold/Controller/Hold Control ==
  FMS_In : Inport
  Action Port : ActionPort  InitializeStates=reset  ActionType=case
  Bus Selector : BusSelector  OutputSignals=INS_Out.psi
  Bus_Selection : Subsystem
  Constant : Constant  Value=0  OutDataTypeStr=Inherit: Inherit via back propagation
  Delay : Delay  DelayLength=1  InitialConditionSource=Input port
      settings: InputPortMap=u0,p4
  Gain2 : Gain  Gain=FMS_PARAM.XY_P  OutDataTypeStr=single
  Multiply : Product  Multiplication=Matrix(*)
  Mux : Mux  Inputs=2
  Psi To DCM : FMT_Model_Lib/Transformation/Psi To DCM
      settings: SourceProductName=FMT Toolbox
  Selector : Selector  InputPortWidth=3  IndexOptions=Index vector (dialog)  Indices=[1 2]  OutputSizes=1
  Sum : Sum  Inputs=-+|
  uv_cmd_mPs : Outport
  wires:
  Bus Selector/1 -> Psi To DCM/1  "<psi>"
  Selector/1 -> Gain2/1
  Mux/1 -> Multiply/2
  Multiply/1 -> Selector/1
  Psi To DCM/1 -> Multiply/1  "M_CO"
  Constant/1 -> Mux/2
  FMS_In/1 -> Bus_Selection/1(FMS_In), Bus Selector/1
  Delay/1 -> Sum/2, Delay/1  "xy_cmd_R"
  Sum/1 -> Mux/1  "xy_err_R"
  Bus_Selection/1(xy_R_O_m) -> Delay/2, Sum/1  "xy_est_R"
  Gain2/1 -> uv_cmd_mPs/1

== system FMS1/FMS Commander/Commander/Arm/SubMode/Hold/Position Hold/Controller/Move Control ==
  FMS_In : Inport
  Action Port : ActionPort  InitializeStates=reset  ActionType=case
  Bus Selector : BusSelector  OutputSignals=Pilot_Cmd.stick_pitch,Pilot_Cmd.stick_roll
  DeadZone : Subsystem  mask{th=FMS_PARAM.PITCH_DZ}
      mask prompts: th "Threshold"
      mask Display: disp('Dead Zone')
  DeadZone1 : Subsystem  mask{th=FMS_PARAM.ROLL_DZ}
      mask prompts: th "Threshold"
      mask Display: disp('Dead Zone')
  Gain6 : Gain  Gain=FMS_PARAM.VEL_XY_LIM  OutDataTypeStr=single
  Mux1 : Mux  Inputs=2
  TD : Subsystem
  uv_cmd_mPs : Outport
  wires:
  Mux1/1 -> Gain6/1
  DeadZone1/1(y) -> Mux1/2
  Bus Selector/2 -> DeadZone1/1(u)  "<stick_roll>"
  TD/1(v1) -> uv_cmd_mPs/1
  FMS_In/1 -> Bus Selector/1
  Bus Selector/1 -> DeadZone/1(u)  "<stick_pitch>"
  DeadZone/1(y) -> Mux1/1
  Gain6/1 -> TD/1(v)

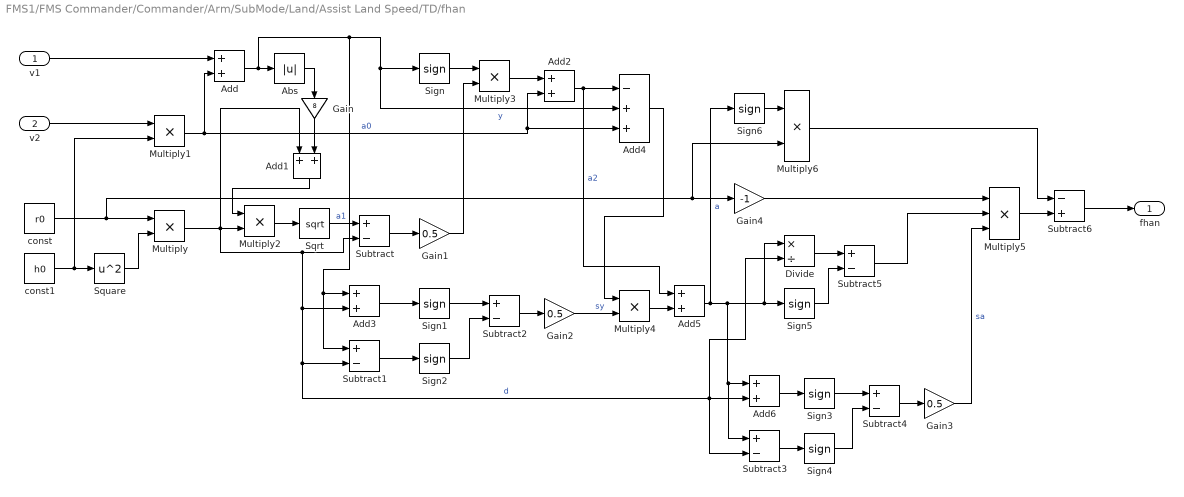
== system FMS1/FMS Commander/Commander/Arm/SubMode/Land/Assist Land Speed/TD/fhan  ==
  v1 : Inport
  v2 : Inport  Port=2
  Abs : Abs
  Add{,1..3,5..6} (6 alike) : Sum  OutDataTypeStr=Inherit: Same as first input
  Add4 : Sum  Inputs=-++
  Divide : Product  Inputs=*/
  Gain : Gain  Gain=8
  Gain1 : Gain  Gain=0.5  OutDataTypeStr=Inherit: Same as input
  Gain2 : Gain  Gain=0.5  OutDataTypeStr=Inherit: Same as input
  Gain3 : Gain  Gain=0.5  OutDataTypeStr=Inherit: Same as input
  Gain4 : Gain  Gain=-1  OutDataTypeStr=Inherit: Same as input
  Multiply{,1..3} (4 alike) : Product  OutDataTypeStr=Inherit: Same as first input
  Multiply4 : Product  OutDataTypeStr=single
  Multiply5 : Product  Inputs=3
  Multiply6 : Product  OutDataTypeStr=single
  Sign{,1..6} (7 alike) : Signum
  Sqrt : Sqrt  SaturateOnIntegerOverflow=on
  Square : Math  Operator=square  SaturateOnIntegerOverflow=on
  Subtract{,1..5} (6 alike) : Sum  Inputs=+-  OutDataTypeStr=Inherit: Same as first input
  Subtract6 : Sum  Inputs=-+  OutDataTypeStr=Inherit: Same as first input
  const : Constant  Value=r0  OutDataTypeStr=single
  const1 : Constant  Value=h0  OutDataTypeStr=single
  fhan : Outport
  wires:
  v1/1 -> Add/1
  Sign/1 -> Multiply3/1
  Gain2/1 -> Multiply4/2  "sy"
  v2/1 -> Multiply1/1
  Gain3/1 -> Multiply5/3  "sa"
  Subtract/1 -> Gain1/1
  Subtract6/1 -> fhan/1
  Sign2/1 -> Subtract2/2
  Sign4/1 -> Subtract4/2
  Abs/1 -> Gain/1
  Add4/1 -> Multiply4/1
  Sign5/1 -> Subtract5/2
  Sqrt/1 -> Subtract/1  "a1"
  Subtract3/1 -> Sign4/1
  Add1/1 -> Multiply2/1
  Subtract1/1 -> Sign2/1
  Divide/1 -> Subtract5/1
  Multiply3/1 -> Add2/1
  Gain/1 -> Add1/2
  const/1 -> Multiply6/2, Gain4/1, Multiply/1
  Add3/1 -> Sign1/1
  Subtract5/1 -> Multiply5/2
  Multiply4/1 -> Add5/2
  const1/1 -> Multiply1/2, Square/1
  Add5/1 -> Sign6/1, Sign5/1, Divide/1, Subtract3/1, Add6/1  "a"
  Multiply1/1 -> Add4/3, Add2/2, Add/2  "a0"
  Add/1 -> Subtract1/1, Add3/1, Add4/2, Sign/1, Abs/1  "y"
  Subtract2/1 -> Gain2/1
  Add2/1 -> Add4/1, Add5/1  "a2"
  Subtract4/1 -> Gain3/1
  Gain4/1 -> Multiply5/1
  Multiply5/1 -> Subtract6/2
  Sign6/1 -> Multiply6/1
  Sign3/1 -> Subtract4/1
  Add6/1 -> Sign3/1
  Multiply/1 -> Subtract/2, Divide/2, Subtract3/2, Add6/2, Subtract1/2, Add3/2, Add1/1, Multiply2/2  "d"
  Multiply6/1 -> Subtract6/1
  Gain1/1 -> Multiply3/2
  Square/1 -> Multiply/2
  Multiply2/1 -> Sqrt/1
  Sign1/1 -> Subtract2/1

== system FMS1/FMS Commander/Commander/Arm/SubMode/Land/Position Command/Position Control/Bus_Selection ==
  FMS_In : Inport
  Bus Selector2 : BusSelector  OutputSignals=INS_Out.x_R,INS_Out.y_R
  Mux : Mux  Inputs=2
  xy_R_O_m : Outport
  wires:
  Bus Selector2/2 -> Mux/2  "<y_R>"
  Mux/1 -> xy_R_O_m/1
  Bus Selector2/1 -> Mux/1  "<x_R>"
  FMS_In/1 -> Bus Selector2/1

== system FMS1/FMS Commander/Commander/Arm/SubMode/Return/Heading Commander/Heading Control/Heading Control ==
  FMS_In : Inport
  psi_cmd_rad : Inport  Port=2
  Bus_Selection : Subsystem
  Gain2 : Gain  Gain=FMS_PARAM.YAW_P  OutDataTypeStr=single
  Saturation : Saturate  UpperLimit=FMS_PARAM.YAW_RATE_LIM  LowerLimit=-FMS_PARAM.YAW_RATE_LIM
  Sum : Sum  Inputs=-+|
  psi_saturation : Subsystem
  psi_rate_cmd_radPs : Outport
  wires:
  Saturation/1 -> psi_rate_cmd_radPs/1
  FMS_In/1 -> Bus_Selection/1(FMS_In)
  Sum/1 -> psi_saturation/1(psi_in)  "psi_error_rad"
  psi_saturation/1(psi_rad) -> Gain2/1
  Bus_Selection/1(psi_rad) -> Sum/1  "psi_est_rad"
  Gain2/1 -> Saturation/1
  psi_cmd_rad/1 -> Sum/2

== system FMS1/FMS Commander/Commander/Arm/SubMode/Return/Heading Commander/Heading Control/TD ==
  v : Inport
  v0 : Inport  Port=2
  Integrator : DiscreteIntegrator  SampleTime=-1  LimitOutput=on  UpperSaturationLimit=FMS_PARAM.YAW_RATE_LIM  LowerSaturationLimit=-FMS_PARAM.YAW_RATE_LIM  ICPrevOutput=DiscIntNeverNeededParam  ICPrevScaledInput=DiscIntNeverNeededParam
  Integrator1 : DiscreteIntegrator  InitialConditionSource=external  SampleTime=-1  ICPrevOutput=DiscIntNeverNeededParam  ICPrevScaledInput=DiscIntNeverNeededParam
  Subtract : Sum  Inputs=+-
  "fhan " : Subsystem  mask{r0=pi/3, h0=pi/4}
      mask DialogControl ParameterGroupVar Prompt: fhan(v1,v2,r0,h0)
  v1 : Outport
  wires:
  Integrator1/1 -> v1/1, Subtract/1
  v/1 -> Subtract/2
  Integrator/1 -> "fhan "/2(v2), Integrator1/1  "v2"
  Subtract/1 -> "fhan "/1(v1)
  "fhan "/1(fhan) -> Integrator/1
  v0/1 -> Integrator1/2

== system FMS1/FMS Commander/Commander/Arm/SubMode/Return/Heading Commander/Heading Control/psi_saturation ==
  psi_in : Inport
  Abs : Abs
  Add : Sum  Inputs=-+
  Compare To Constant : simulink/Logic and Bit Operations/Compare To Constant  relop=>  const=pi  OutDataTypeStr=boolean
  Constant : Constant  Value=2*pi  OutDataTypeStr=single
  Constant1 : Constant  Value=2*pi  OutDataTypeStr=single
  Multiply : Product
  Rem : Math  Operator=rem  SaturateOnIntegerOverflow=on
  Sign : Signum
  Switch : Switch  Criteria=u2 > Threshold
  psi_rad : Outport
  wires:
  Constant1/1 -> Rem/2
  psi_in/1 -> Rem/1
  Switch/1 -> psi_rad/1
  Sign/1 -> Multiply/2
  Constant/1 -> Multiply/1
  Multiply/1 -> Add/1
  Add/1 -> Switch/1
  Compare To Constant/1 -> Switch/2
  Abs/1 -> Compare To Constant/1
  Rem/1 -> Abs/1, Switch/3, Add/2, Sign/1

== system FMS1/FMS Commander/Commander/Arm/SubMode/Return/Heading Commander/Heading Control/psi_saturation1 ==
  psi_in : Inport
  Abs : Abs
  Add : Sum  Inputs=-+
  Compare To Constant : simulink/Logic and Bit Operations/Compare To Constant  relop=>  const=pi  OutDataTypeStr=boolean
  Constant : Constant  Value=2*pi  OutDataTypeStr=single
  Constant1 : Constant  Value=2*pi  OutDataTypeStr=single
  Multiply : Product
  Rem : Math  Operator=rem  SaturateOnIntegerOverflow=on
  Sign : Signum
  Switch : Switch  Criteria=u2 > Threshold
  psi_rad : Outport
  wires:
  Rem/1 -> Sign/1, Add/2, Switch/3, Abs/1
  Abs/1 -> Compare To Constant/1
  Compare To Constant/1 -> Switch/2
  Add/1 -> Switch/1
  Multiply/1 -> Add/1
  Constant/1 -> Multiply/1
  Sign/1 -> Multiply/2
  Switch/1 -> psi_rad/1
  psi_in/1 -> Rem/1
  Constant1/1 -> Rem/2

== system FMS1/FMS Commander/Commander/Arm/SubMode/Return/Velocity Commander1/Altitude Control/Target Height ==
  FMS_In : Inport
  Add : Sum
  Bus Selector : BusSelector  OutputSignals=Cmd_In.sp_waypoint,Cmd_In.cur_waypoint
  Bus Selector1 : BusSelector  OutputSignals=INS_Out.x_R,INS_Out.y_R
  Bus Selector2 : BusSelector  OutputSignals=Cmd_In.cur_waypoint,Cmd_In.sp_waypoint
  Divide : Product  Inputs=*/
  Multiply : Product
  Mux : Mux  Inputs=2
  Saturation : Saturate  UpperLimit=1  LowerLimit=0
  Selector : Selector  InputPortWidth=3  IndexOptions=Index vector (dialog)  Indices=3  OutputSizes=1
  Selector1 : Selector  InputPortWidth=3  IndexOptions=Index vector (dialog)  Indices=3  OutputSizes=1
  Selector2 : Selector  InputPortWidth=3  IndexOptions=Index vector (dialog)  Indices=[1 2]  OutputSizes=1
  Selector3 : Selector  InputPortWidth=3  IndexOptions=Index vector (dialog)  Indices=[1 2]  OutputSizes=1
  Subtract : Sum  Inputs=+-
  Sum : Sum  Inputs=|+-
  Sum1 : Sum  Inputs=-+|
  Vector Modulus : FMT_Model_Lib/Math/Vector Modulus
      settings: SourceProductName=FMT Toolbox
  Vector Modulus1 : FMT_Model_Lib/Math/Vector Modulus
      settings: SourceProductName=FMT Toolbox
  h_R_sp : Outport
  wires:
  Multiply/1 -> Add/2
  Bus Selector1/1 -> Mux/1  "<x_R>"
  Bus Selector/1 -> Selector1/1  "<sp_waypoint>"
  Vector Modulus1/1 -> Divide/2
  Sum1/1 -> Vector Modulus1/1
  Sum/1 -> Vector Modulus/1
  Selector2/1 -> Sum1/1, Sum/2
  FMS_In/1 -> Bus Selector2/1, Bus Selector1/1, Bus Selector/1
  Bus Selector2/2 -> Selector3/1  "<sp_waypoint>"
  Vector Modulus/1 -> Divide/1
  Bus Selector1/2 -> Mux/2  "<y_R>"
  Bus Selector2/1 -> Selector2/1  "<cur_waypoint>"
  Selector1/1 -> Subtract/1
  Mux/1 -> Sum/1
  Subtract/1 -> Multiply/1
  Divide/1 -> Saturation/1
  Selector3/1 -> Sum1/2
  Bus Selector/2 -> Selector/1  "<cur_waypoint>"
  Selector/1 -> Add/1, Subtract/2
  Saturation/1 -> Multiply/2
  Add/1 -> h_R_sp/1

== system FMS1/FMS Commander/Commander/Arm/SubMode/Return/Velocity Commander1/Hold Position/Altitude Hold ==
  FMS_In : Inport
  Controller : Subsystem
  Detect Movement : Subsystem
  w_cmd_mPs : Outport
  wires:
  Controller/1(w_cmd_mPs) -> w_cmd_mPs/1
  Detect Movement/1(motion_state) -> Controller/1(motion_state)
  FMS_In/1 -> Controller/2(FMS_In), Detect Movement/1(FMS_In)

== system FMS1/FMS Commander/Commander/Arm/SubMode/Return/Velocity Commander1/Hold Position/Position Hold ==
  FMS_In : Inport
  Controller : Subsystem
  Demux : Demux  Outputs=2
  Detect Movement : Subsystem
  u_cmd_mPs : Outport
  v_cmd_mPs : Outport  Port=2
  wires:
  FMS_In/1 -> Controller/2(FMS_In), Detect Movement/1(FMS_In)
  Demux/2 -> v_cmd_mPs/1
  Demux/1 -> u_cmd_mPs/1
  Controller/1(uv_cmd_mPs) -> Demux/1
  Detect Movement/1(motion_state) -> Controller/1(motion_state)

== system FMS1/FMS Commander/Commander/Arm/SubMode/Return/Velocity Commander1/Lateral Acceleration/Included Angle ==
  vec1 : Inport
  vec2 : Inport  Port=2
  2D Cross Product : FMT_Model_Lib/Math/2D Cross Product
      settings: SourceProductName=FMT Toolbox
  Acos : Trigonometry  Operator=acos
  Constant4 : Constant  OutDataTypeStr=single
  Demux : Demux  Outputs=2
  Demux1 : Demux  Outputs=2
  Dot Product : DotProduct  InputSameDT=on  OutDataTypeStr=Inherit: Inherit via internal rule
  Multiply : Product
  Mux : Mux  Inputs=2
  Mux1 : Mux  Inputs=2
  Sign1 : Signum
  Switch2 : Switch  Criteria=u2 ~= 0
  Vector Normalize : FMT_Model_Lib/Math/Vector Normalize
      settings: SourceProductName=FMT Toolbox
  Vector Normalize1 : FMT_Model_Lib/Math/Vector Normalize
      settings: SourceProductName=FMT Toolbox
  angle_rad : Outport
  wires:
  Switch2/1 -> Multiply/2
  Acos/1 -> Multiply/1
  Mux/1 -> Vector Normalize1/1
  vec2/1 -> Demux/1
  Constant4/1 -> Switch2/3
  Demux/1 -> Mux/2
  vec1/1 -> Demux1/1
  Multiply/1 -> angle_rad/1
  2D Cross Product/1 -> Sign1/1
  Vector Normalize/1 -> 2D Cross Product/2, Dot Product/1
  Demux/2 -> Mux/1
  Vector Normalize1/1 -> 2D Cross Product/1, Dot Product/2
  Sign1/1 -> Switch2/2, Switch2/1
  Demux1/2 -> Mux1/1
  Mux1/1 -> Vector Normalize/1
  Demux1/1 -> Mux1/2
  Dot Product/1 -> Acos/1

== system FMS1/FMS Commander/Commander/Arm/SubMode/Return/Velocity Commander1/Lateral Acceleration To Speed/Ground Speed ==
  |Vg| : Inport
  p3p2 : Inport  Port=2
  Constant : Constant  Value=0  OutDataTypeStr=single
  Multiply2 : Product
  Mux : Mux  Inputs=2
  Vector Normalize2 : FMT_Model_Lib/Math/Vector Normalize
      settings: SourceProductName=FMT Toolbox
  Vg_O_cmd : Outport
  wires:
  |Vg|/1 -> Multiply2/2
  Constant/1 -> Mux/2
  Mux/1 -> Vector Normalize2/1
  p3p2/1 -> Mux/1
  Vector Normalize2/1 -> Multiply2/1
  Multiply2/1 -> Vg_O_cmd/1

== system FMS1/FMS Commander/Commander/Arm/SubMode/Return/Velocity Commander1/Lateral Acceleration To Speed/Rotation Matrix ==
  l1_omega : Inport
  psi : Inport  Port=2
  Add : Sum  Inputs=-+
  Discrete-Time Integrator : DiscreteIntegrator  SampleTime=-1  StateName=l1_heading  ICPrevOutput=DiscIntNeverNeededParam  ICPrevScaledInput=DiscIntNeverNeededParam
  Psi To DCM : FMT_Model_Lib/Transformation/Psi To DCM
      settings: SourceProductName=FMT Toolbox
  M_CO : Outport
  wires:
  Add/1 -> Psi To DCM/1
  l1_omega/1 -> Discrete-Time Integrator/1  "l1_omega"
  psi/1 -> Add/2
  Discrete-Time Integrator/1 -> Add/1  "l1_psi"
  Psi To DCM/1 -> M_CO/1

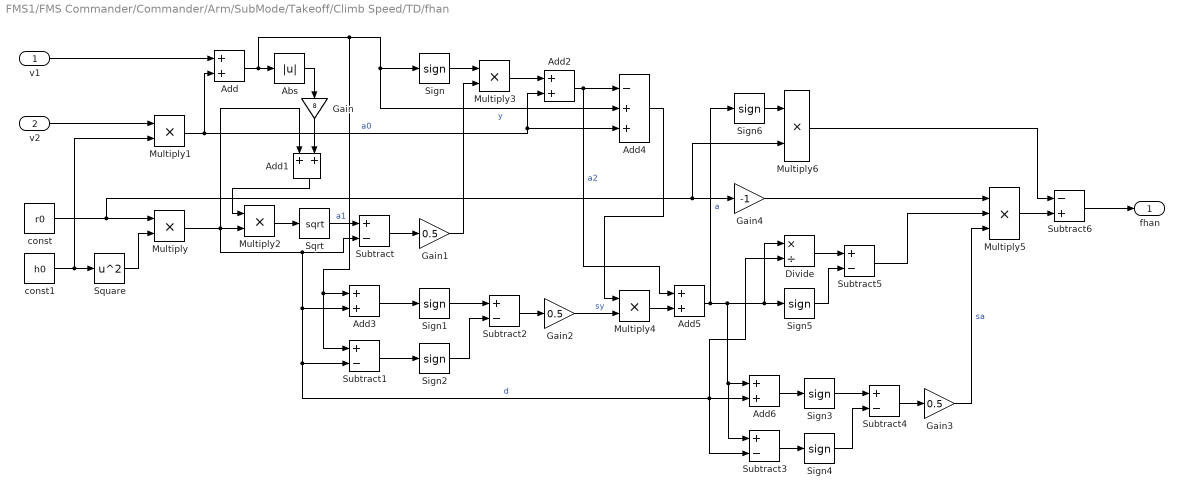
== system FMS1/FMS Commander/Commander/Arm/SubMode/Takeoff/Climb Speed/TD/fhan  ==
  v1 : Inport
  v2 : Inport  Port=2
  Abs : Abs
  Add{,1..3,5..6} (6 alike) : Sum  OutDataTypeStr=Inherit: Same as first input
  Add4 : Sum  Inputs=-++
  Divide : Product  Inputs=*/
  Gain : Gain  Gain=8
  Gain1 : Gain  Gain=0.5  OutDataTypeStr=Inherit: Same as input
  Gain2 : Gain  Gain=0.5  OutDataTypeStr=Inherit: Same as input
  Gain3 : Gain  Gain=0.5  OutDataTypeStr=Inherit: Same as input
  Gain4 : Gain  Gain=-1  OutDataTypeStr=Inherit: Same as input
  Multiply{,1..3} (4 alike) : Product  OutDataTypeStr=Inherit: Same as first input
  Multiply4 : Product  OutDataTypeStr=single
  Multiply5 : Product  Inputs=3
  Multiply6 : Product  OutDataTypeStr=single
  Sign{,1..6} (7 alike) : Signum
  Sqrt : Sqrt  SaturateOnIntegerOverflow=on
  Square : Math  Operator=square  SaturateOnIntegerOverflow=on
  Subtract{,1..5} (6 alike) : Sum  Inputs=+-  OutDataTypeStr=Inherit: Same as first input
  Subtract6 : Sum  Inputs=-+  OutDataTypeStr=Inherit: Same as first input
  const : Constant  Value=r0  OutDataTypeStr=single
  const1 : Constant  Value=h0  OutDataTypeStr=single
  fhan : Outport
  wires:
  v1/1 -> Add/1
  Sign/1 -> Multiply3/1
  Gain2/1 -> Multiply4/2  "sy"
  v2/1 -> Multiply1/1
  Gain3/1 -> Multiply5/3  "sa"
  Subtract/1 -> Gain1/1
  Subtract6/1 -> fhan/1
  Sign2/1 -> Subtract2/2
  Sign4/1 -> Subtract4/2
  Abs/1 -> Gain/1
  Add4/1 -> Multiply4/1
  Sign5/1 -> Subtract5/2
  Sqrt/1 -> Subtract/1  "a1"
  Subtract3/1 -> Sign4/1
  Add1/1 -> Multiply2/1
  Subtract1/1 -> Sign2/1
  Divide/1 -> Subtract5/1
  Multiply3/1 -> Add2/1
  Gain/1 -> Add1/2
  const/1 -> Multiply6/2, Gain4/1, Multiply/1
  Add3/1 -> Sign1/1
  Subtract5/1 -> Multiply5/2
  Multiply4/1 -> Add5/2
  const1/1 -> Multiply1/2, Square/1
  Add5/1 -> Sign6/1, Sign5/1, Divide/1, Subtract3/1, Add6/1  "a"
  Multiply1/1 -> Add4/3, Add2/2, Add/2  "a0"
  Add/1 -> Subtract1/1, Add3/1, Add4/2, Sign/1, Abs/1  "y"
  Subtract2/1 -> Gain2/1
  Add2/1 -> Add4/1, Add5/1  "a2"
  Subtract4/1 -> Gain3/1
  Gain4/1 -> Multiply5/1
  Multiply5/1 -> Subtract6/2
  Sign6/1 -> Multiply6/1
  Sign3/1 -> Subtract4/1
  Add6/1 -> Sign3/1
  Multiply/1 -> Subtract/2, Divide/2, Subtract3/2, Add6/2, Subtract1/2, Add3/2, Add1/1, Multiply2/2  "d"
  Multiply6/1 -> Subtract6/1
  Gain1/1 -> Multiply3/2
  Square/1 -> Multiply/2
  Multiply2/1 -> Sqrt/1
  Sign1/1 -> Subtract2/1

== system FMS1/FMS Commander/Commander/Arm/Assist/Altitude/Altitude Command/Controller/Hold Control/Bus_Selection ==
  FMS_In : Inport
  Bus Selector2 : BusSelector  OutputSignals=INS_Out.h_R
  Gain : Gain  Gain=-1
  z_R_m : Outport
  wires:
  Gain/1 -> z_R_m/1
  Bus Selector2/1 -> Gain/1  "<h_R>"
  FMS_In/1 -> Bus Selector2/1

== system FMS1/FMS Commander/Commander/Arm/Assist/Altitude/Altitude Command/Controller/Move Control/Assist Land Speed ==
  u : Inport
  Gain : Gain  Gain=0.5
  Land_Speed : Constant  Value=FMS_PARAM.LAND_SPEED  OutDataTypeStr=single
  Min : MinMax  Inputs=2
  y : Outport
  wires:
  u/1 -> Min/2
  Land_Speed/1 -> Min/1
  Min/1 -> Gain/1
  Gain/1 -> y/1
